simulink library "FilterLib"  (R2018a)
settings: Solver=VariableStepAuto  StartTime=0.0  StopTime=10.0  RelTol=1e-3
settings Model: Creator=Ismail Shaikh  LastModifiedBy=Ismail Shaikh

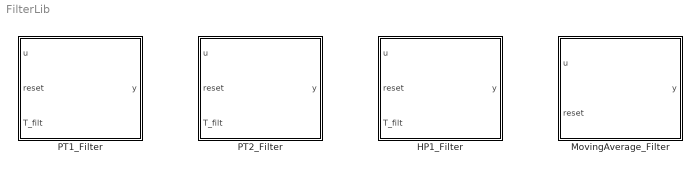
== system FilterLib ==
  HP1_Filter : Subsystem  mask(HP1 Filter){Ts=0.01, Method=Forward Euler: K = Ts/T, y0=0}
      mask prompts: Ts "Task time Ts [s]"; Method "Discretisation method"; y0 "Initial low-pass state y0"
      mask help: Discrete 1st-order high pass: y = u - PT1(u). Passes changes, removes the steady part. reset ~= 0 sets y = 0.
      mask init:
      | if ~(isscalar(Ts) && isfinite(Ts) && Ts > 0), error('Task time Ts must be a positive, finite scalar.'); end
      mask TypeOptions Method: Forward Euler: K = Ts/T | Backward Euler: K = Ts/(T+Ts) | Exact: K = 1-exp(-Ts/T)
      mask Display:
      | disp('HP1');
      | port_label('input',1,'u');
      | port_label('input',2,'reset');
      | port_label('input',3,'T_filt');
      | port_label('output',1,'y');
  MovingAverage_Filter : Subsystem  mask(Moving Average Filter){N=10, y0=0}
      mask prompts: N "Window length N [samples]"; y0 "Initial output y0"
      mask help: FIR filter: y = mean of the last N input samples. reset ~= 0 fills the window with u (y = u).
      mask init:
      | if ~(isscalar(N) && N >= 1 && N == round(N)), error('Window length N must be an integer >= 1.'); end
      mask Display:
      | disp('MovAvg');
      | port_label('input',1,'u');
      | port_label('input',2,'reset');
      | port_label('output',1,'y');
  PT1_Filter : Subsystem  mask(PT1 Filter){Ts=0.01, Method=Forward Euler: K = Ts/T, y0=0}
      mask prompts: Ts "Task time Ts [s]"; Method "Discretisation method"; y0 "Initial output y0"
      mask help: Discrete 1st-order low pass. y = y_prev + K*(u - y_prev). reset ~= 0 sets y = u.
      mask init:
      | if ~(isscalar(Ts) && isfinite(Ts) && Ts > 0), error('Task time Ts must be a positive, finite scalar.'); end
      mask TypeOptions Method: Forward Euler: K = Ts/T | Backward Euler: K = Ts/(T+Ts) | Exact: K = 1-exp(-Ts/T)
      mask Display:
      | disp('PT1');
      | port_label('input',1,'u');
      | port_label('input',2,'reset');
      | port_label('input',3,'T_filt');
      | port_label('output',1,'y');
  PT2_Filter : Subsystem  mask(PT2 Filter){Ts=0.01, Method=Forward Euler: K = Ts/T, y0=0}
      mask prompts: Ts "Task time Ts [s]"; Method "Discretisation method"; y0 "Initial output y0 (both stages)"
      mask help: Two identical PT1 stages in series (critically damped 2nd-order low pass), each with time constant T_filt. reset ~= 0 sets y = u.
      mask init:
      | if ~(isscalar(Ts) && isfinite(Ts) && Ts > 0), error('Task time Ts must be a positive, finite scalar.'); end
      mask TypeOptions Method: Forward Euler: K = Ts/T | Backward Euler: K = Ts/(T+Ts) | Exact: K = 1-exp(-Ts/T)
      mask Display:
      | disp('PT2');
      | port_label('input',1,'u');
      | port_label('input',2,'reset');
      | port_label('input',3,'T_filt');
      | port_label('output',1,'y');

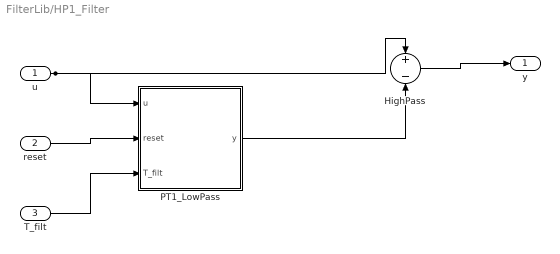
== system FilterLib/HP1_Filter ==
  u : Inport
  reset : Inport  Port=2
  T_filt : Inport  Port=3
  HighPass : Sum  Inputs=+-
  PT1_LowPass : Subsystem
  y : Outport
  wires:
  u/1 -> PT1_LowPass/1(u), HighPass/1
  reset/1 -> PT1_LowPass/2(reset)
  T_filt/1 -> PT1_LowPass/3(T_filt)
  PT1_LowPass/1(y) -> HighPass/2
  HighPass/1 -> y/1

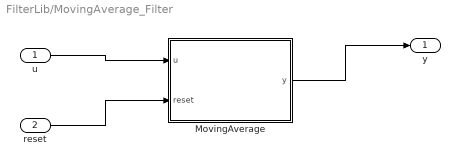
== system FilterLib/MovingAverage_Filter ==
  u : Inport
  reset : Inport  Port=2
  MovingAverage : MATLAB Function  TreatAsAtomicUnit=on
  y : Outport
  wires:
  u/1 -> MovingAverage/1(u)
  reset/1 -> MovingAverage/2(reset)
  MovingAverage/1(y) -> y/1

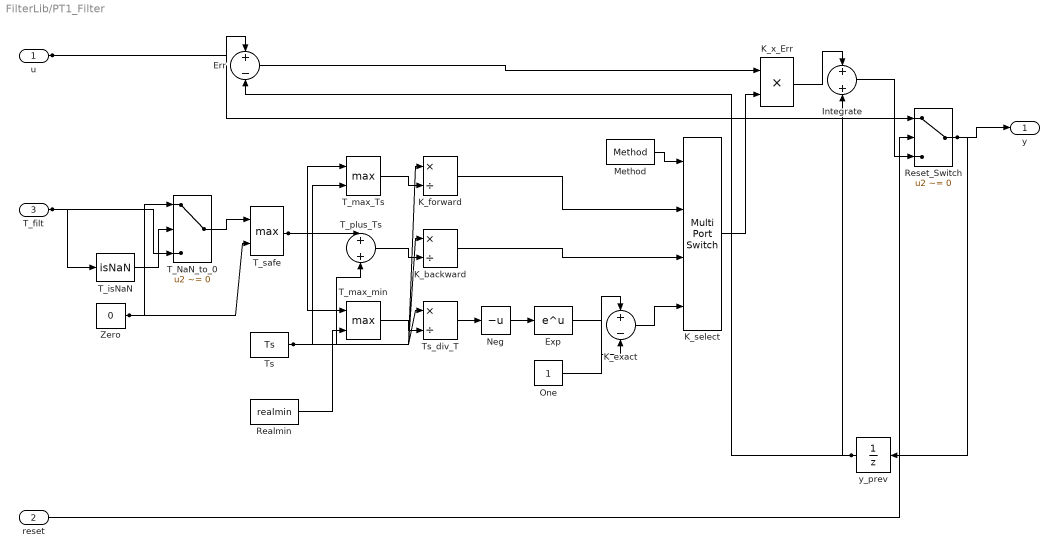
== system FilterLib/PT1_Filter ==
  u : Inport
  reset : Inport  Port=2
  T_filt : Inport  Port=3
  Err : Sum  Inputs=+-
  Exp : Math  SaturateOnIntegerOverflow=on
  Integrate : Sum
  K_backward : Product  Inputs=*/
  K_exact : Sum  Inputs=+-
  K_forward : Product  Inputs=*/
  K_select : MultiPortSwitch
  K_x_Err : Product
  Method : Constant  Value=Method
  Neg : UnaryMinus
  One : Constant
  Realmin : Constant  Value=realmin
  Reset_Switch : Switch  Criteria=u2 ~= 0
  T_NaN_to_0 : Switch  Criteria=u2 ~= 0
  T_isNaN : RelationalOperator  Operator=isNaN  OutDataTypeStr=boolean  RndMeth=Simplest
  T_max_Ts : MinMax  Function=max  Inputs=2
  T_max_min : MinMax  Function=max  Inputs=2
  T_plus_Ts : Sum
  T_safe : MinMax  Function=max  Inputs=2
  Ts : Constant  Value=Ts
  Ts_div_T : Product  Inputs=*/
  Zero : Constant  Value=0
  y_prev : UnitDelay  InitialCondition=y0  SampleTime=-1
  y : Outport
  wires:
  T_filt/1 -> T_isNaN/1, T_NaN_to_0/3
  Zero/1 -> T_NaN_to_0/1, T_safe/2
  T_isNaN/1 -> T_NaN_to_0/2
  T_NaN_to_0/1 -> T_safe/1
  T_safe/1 -> T_max_Ts/1, T_plus_Ts/1, T_max_min/1
  Ts/1 -> T_max_Ts/2, K_forward/1, T_plus_Ts/2, K_backward/1, Ts_div_T/1
  T_max_Ts/1 -> K_forward/2
  T_plus_Ts/1 -> K_backward/2
  Realmin/1 -> T_max_min/2
  T_max_min/1 -> Ts_div_T/2
  Ts_div_T/1 -> Neg/1
  Neg/1 -> Exp/1
  One/1 -> K_exact/1
  Exp/1 -> K_exact/2
  Method/1 -> K_select/1
  K_forward/1 -> K_select/2
  K_backward/1 -> K_select/3
  K_exact/1 -> K_select/4
  u/1 -> Err/1, Reset_Switch/1
  y_prev/1 -> Err/2, Integrate/2
  Err/1 -> K_x_Err/1
  K_select/1 -> K_x_Err/2
  K_x_Err/1 -> Integrate/1
  reset/1 -> Reset_Switch/2
  Integrate/1 -> Reset_Switch/3
  Reset_Switch/1 -> y/1, y_prev/1

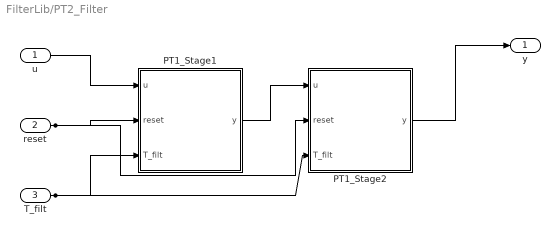
== system FilterLib/PT2_Filter ==
  u : Inport
  reset : Inport  Port=2
  T_filt : Inport  Port=3
  PT1_Stage1 : Subsystem
  PT1_Stage2 : Subsystem
  y : Outport
  wires:
  u/1 -> PT1_Stage1/1(u)
  reset/1 -> PT1_Stage1/2(reset), PT1_Stage2/2(reset)
  T_filt/1 -> PT1_Stage1/3(T_filt), PT1_Stage2/3(T_filt)
  PT1_Stage1/1(y) -> PT1_Stage2/1(u)
  PT1_Stage2/1(y) -> y/1

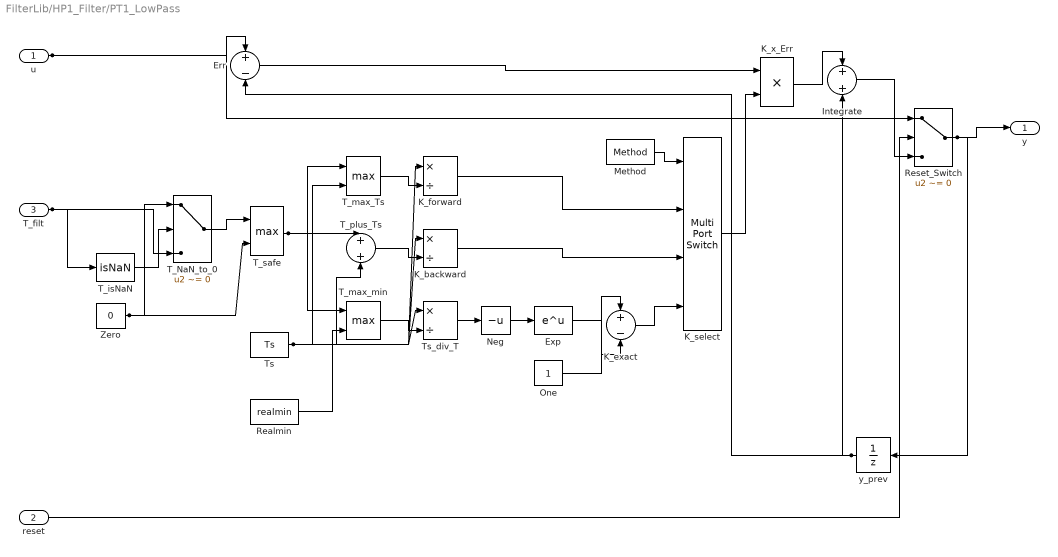
== system FilterLib/HP1_Filter/PT1_LowPass ==
  u : Inport
  reset : Inport  Port=2
  T_filt : Inport  Port=3
  Err : Sum  Inputs=+-
  Exp : Math  SaturateOnIntegerOverflow=on
  Integrate : Sum
  K_backward : Product  Inputs=*/
  K_exact : Sum  Inputs=+-
  K_forward : Product  Inputs=*/
  K_select : MultiPortSwitch
  K_x_Err : Product
  Method : Constant  Value=Method
  Neg : UnaryMinus
  One : Constant
  Realmin : Constant  Value=realmin
  Reset_Switch : Switch  Criteria=u2 ~= 0
  T_NaN_to_0 : Switch  Criteria=u2 ~= 0
  T_isNaN : RelationalOperator  Operator=isNaN  OutDataTypeStr=boolean  RndMeth=Simplest
  T_max_Ts : MinMax  Function=max  Inputs=2
  T_max_min : MinMax  Function=max  Inputs=2
  T_plus_Ts : Sum
  T_safe : MinMax  Function=max  Inputs=2
  Ts : Constant  Value=Ts
  Ts_div_T : Product  Inputs=*/
  Zero : Constant  Value=0
  y_prev : UnitDelay  InitialCondition=y0  SampleTime=-1
  y : Outport
  wires:
  T_filt/1 -> T_isNaN/1, T_NaN_to_0/3
  Zero/1 -> T_NaN_to_0/1, T_safe/2
  T_isNaN/1 -> T_NaN_to_0/2
  T_NaN_to_0/1 -> T_safe/1
  T_safe/1 -> T_max_Ts/1, T_plus_Ts/1, T_max_min/1
  Ts/1 -> T_max_Ts/2, K_forward/1, T_plus_Ts/2, K_backward/1, Ts_div_T/1
  T_max_Ts/1 -> K_forward/2
  T_plus_Ts/1 -> K_backward/2
  Realmin/1 -> T_max_min/2
  T_max_min/1 -> Ts_div_T/2
  Ts_div_T/1 -> Neg/1
  Neg/1 -> Exp/1
  One/1 -> K_exact/1
  Exp/1 -> K_exact/2
  Method/1 -> K_select/1
  K_forward/1 -> K_select/2
  K_backward/1 -> K_select/3
  K_exact/1 -> K_select/4
  u/1 -> Err/1, Reset_Switch/1
  y_prev/1 -> Err/2, Integrate/2
  Err/1 -> K_x_Err/1
  K_select/1 -> K_x_Err/2
  K_x_Err/1 -> Integrate/1
  reset/1 -> Reset_Switch/2
  Integrate/1 -> Reset_Switch/3
  Reset_Switch/1 -> y/1, y_prev/1

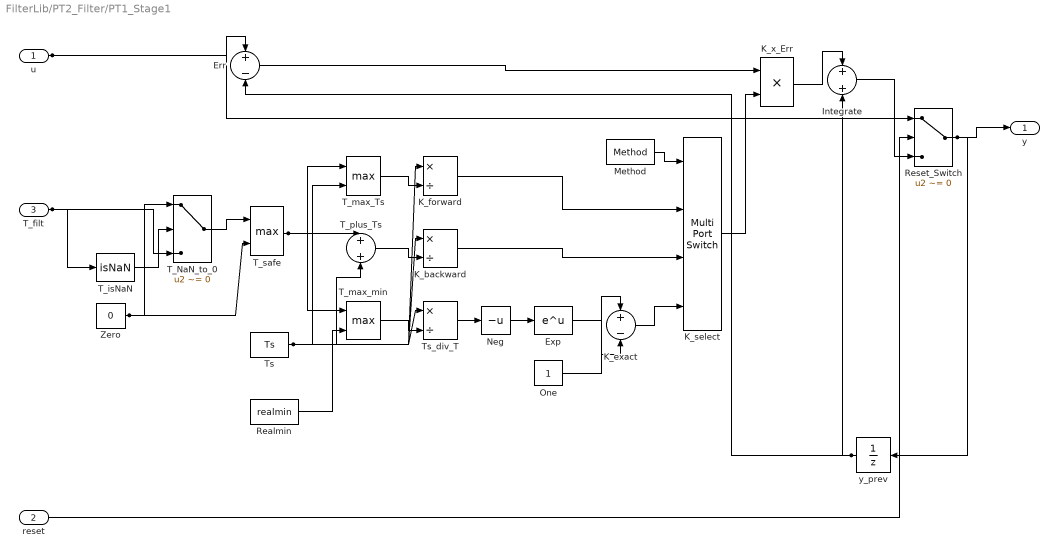
== system FilterLib/PT2_Filter/PT1_Stage1 ==
  u : Inport
  reset : Inport  Port=2
  T_filt : Inport  Port=3
  Err : Sum  Inputs=+-
  Exp : Math  SaturateOnIntegerOverflow=on
  Integrate : Sum
  K_backward : Product  Inputs=*/
  K_exact : Sum  Inputs=+-
  K_forward : Product  Inputs=*/
  K_select : MultiPortSwitch
  K_x_Err : Product
  Method : Constant  Value=Method
  Neg : UnaryMinus
  One : Constant
  Realmin : Constant  Value=realmin
  Reset_Switch : Switch  Criteria=u2 ~= 0
  T_NaN_to_0 : Switch  Criteria=u2 ~= 0
  T_isNaN : RelationalOperator  Operator=isNaN  OutDataTypeStr=boolean  RndMeth=Simplest
  T_max_Ts : MinMax  Function=max  Inputs=2
  T_max_min : MinMax  Function=max  Inputs=2
  T_plus_Ts : Sum
  T_safe : MinMax  Function=max  Inputs=2
  Ts : Constant  Value=Ts
  Ts_div_T : Product  Inputs=*/
  Zero : Constant  Value=0
  y_prev : UnitDelay  InitialCondition=y0  SampleTime=-1
  y : Outport
  wires:
  T_filt/1 -> T_isNaN/1, T_NaN_to_0/3
  Zero/1 -> T_NaN_to_0/1, T_safe/2
  T_isNaN/1 -> T_NaN_to_0/2
  T_NaN_to_0/1 -> T_safe/1
  T_safe/1 -> T_max_Ts/1, T_plus_Ts/1, T_max_min/1
  Ts/1 -> T_max_Ts/2, K_forward/1, T_plus_Ts/2, K_backward/1, Ts_div_T/1
  T_max_Ts/1 -> K_forward/2
  T_plus_Ts/1 -> K_backward/2
  Realmin/1 -> T_max_min/2
  T_max_min/1 -> Ts_div_T/2
  Ts_div_T/1 -> Neg/1
  Neg/1 -> Exp/1
  One/1 -> K_exact/1
  Exp/1 -> K_exact/2
  Method/1 -> K_select/1
  K_forward/1 -> K_select/2
  K_backward/1 -> K_select/3
  K_exact/1 -> K_select/4
  u/1 -> Err/1, Reset_Switch/1
  y_prev/1 -> Err/2, Integrate/2
  Err/1 -> K_x_Err/1
  K_select/1 -> K_x_Err/2
  K_x_Err/1 -> Integrate/1
  reset/1 -> Reset_Switch/2
  Integrate/1 -> Reset_Switch/3
  Reset_Switch/1 -> y/1, y_prev/1

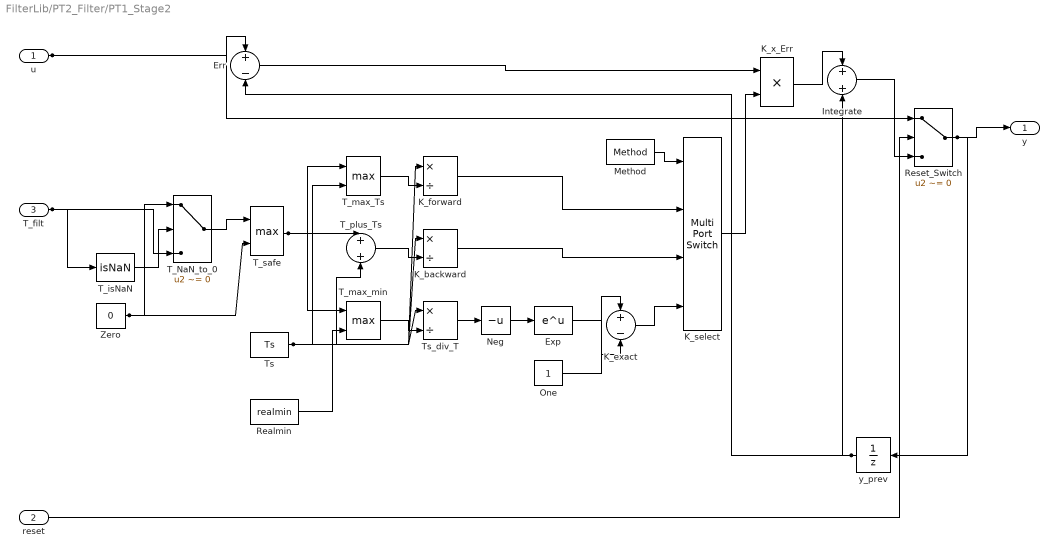
== system FilterLib/PT2_Filter/PT1_Stage2 ==
  u : Inport
  reset : Inport  Port=2
  T_filt : Inport  Port=3
  Err : Sum  Inputs=+-
  Exp : Math  SaturateOnIntegerOverflow=on
  Integrate : Sum
  K_backward : Product  Inputs=*/
  K_exact : Sum  Inputs=+-
  K_forward : Product  Inputs=*/
  K_select : MultiPortSwitch
  K_x_Err : Product
  Method : Constant  Value=Method
  Neg : UnaryMinus
  One : Constant
  Realmin : Constant  Value=realmin
  Reset_Switch : Switch  Criteria=u2 ~= 0
  T_NaN_to_0 : Switch  Criteria=u2 ~= 0
  T_isNaN : RelationalOperator  Operator=isNaN  OutDataTypeStr=boolean  RndMeth=Simplest
  T_max_Ts : MinMax  Function=max  Inputs=2
  T_max_min : MinMax  Function=max  Inputs=2
  T_plus_Ts : Sum
  T_safe : MinMax  Function=max  Inputs=2
  Ts : Constant  Value=Ts
  Ts_div_T : Product  Inputs=*/
  Zero : Constant  Value=0
  y_prev : UnitDelay  InitialCondition=y0  SampleTime=-1
  y : Outport
  wires:
  T_filt/1 -> T_isNaN/1, T_NaN_to_0/3
  Zero/1 -> T_NaN_to_0/1, T_safe/2
  T_isNaN/1 -> T_NaN_to_0/2
  T_NaN_to_0/1 -> T_safe/1
  T_safe/1 -> T_max_Ts/1, T_plus_Ts/1, T_max_min/1
  Ts/1 -> T_max_Ts/2, K_forward/1, T_plus_Ts/2, K_backward/1, Ts_div_T/1
  T_max_Ts/1 -> K_forward/2
  T_plus_Ts/1 -> K_backward/2
  Realmin/1 -> T_max_min/2
  T_max_min/1 -> Ts_div_T/2
  Ts_div_T/1 -> Neg/1
  Neg/1 -> Exp/1
  One/1 -> K_exact/1
  Exp/1 -> K_exact/2
  Method/1 -> K_select/1
  K_forward/1 -> K_select/2
  K_backward/1 -> K_select/3
  K_exact/1 -> K_select/4
  u/1 -> Err/1, Reset_Switch/1
  y_prev/1 -> Err/2, Integrate/2
  Err/1 -> K_x_Err/1
  K_select/1 -> K_x_Err/2
  K_x_Err/1 -> Integrate/1
  reset/1 -> Reset_Switch/2
  Integrate/1 -> Reset_Switch/3
  Reset_Switch/1 -> y/1, y_prev/1

== matlab function FilterLib/MovingAverage_Filter/MovingAverage ==
  data: u input; y output; reset input; N parameter; y0 parameter
function y = MovingAverage(u, reset, N, y0)
%#codegen
% Average of the last N samples (circular buffer).
% sum(buf) is recomputed every step: no drift from a running sum.
persistent buf k
if isempty(buf)
    buf = y0 * ones(N, 1);
    k = 1;
end
if reset ~= 0
    buf(:) = u;          % reset: fill window with current input -> y = u
else
    buf(k) = u;
    k = k + 1;
    if k > N, k = 1; end
end
y = sum(buf) / N;
